simulink model "TotemPoleBoostPFCTestHarnessPlant"  (R2026a)
settings: Solver=ode3  StopTime=0.08  MaxStep=1e-5  AbsTol=1e-3
PreLoadFcn:
  | TotemPoleBoostPFCDefaultInputParameters;
model workspace (MAT data in the model file):
  ConverterKey = "TotemPoleBoostPFC"
undefined symbols (not defined in the file or in its folder): DiscIntNeverNeededParam, totemPoleController, totemPoleDesign
libraries: ee_lib x27, nesl_utility x23, fl_lib x12
(part 1 of 3)
settings Model: Creator=vsolaise  LastModifiedBy=vsolaise
settings SimscapeCC: SimscapeNominalValues="[{\"value\":\"1\",\"unit\":\"A\"},{\"value\":\"1\",\"unit\":\"bar\"},{\"value\":\"1\",\"unit\":\"cm^2\"},{\"value\":\"1\",\"unit\":\"cm^3/s\"},{\"value\":\"1\",\"unit\":\"kJ/kg\"},{\"value\":\"1\",\"unit\":\"kW\"},{\"value\":\"1\",\"unit\":\"l\"},{\"value\":\"1\",\"unit\":\"N\"},{\"value\":\"1\",\"unit\":\"N*m\"},{\"value\":\"1\",\"unit\":\"V\"}]"  SimscapeLogDataHistory=5000.0

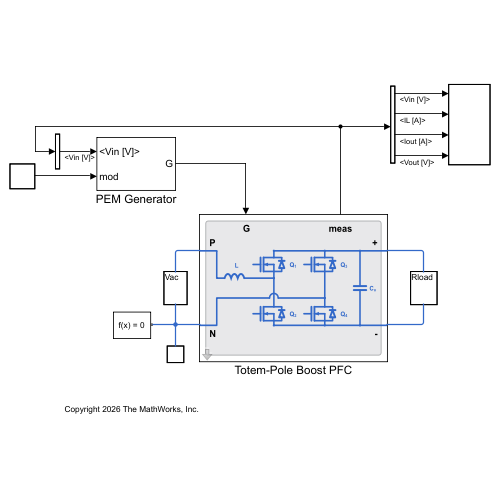
[thumbnail: Simulink's stored preview of the top-level diagram]
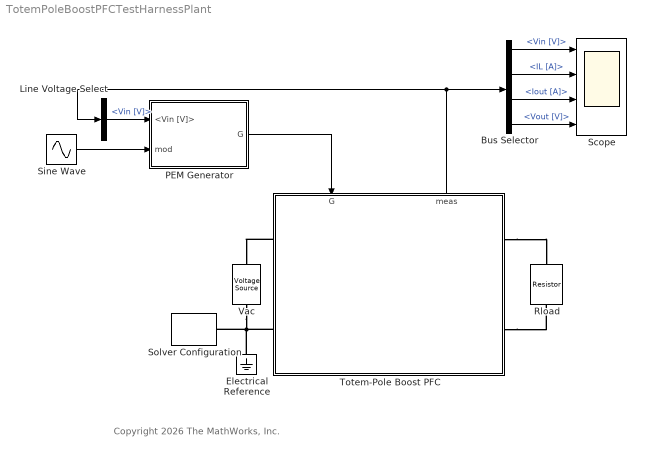
== system TotemPoleBoostPFCTestHarnessPlant ==
  note: Copyright 2026 The MathWorks, Inc.
  Bus Selector : BusSelector  OutputSignals=Vin [V],IL [A],Iout [A],Vout [V]
  Electrical Reference : fl_lib/Electrical/Electrical Elements/Electrical Reference
  Line Voltage Select : BusSelector  OutputSignals=Vin [V]
  PEM Generator : Subsystem
  Rload : fl_lib/Electrical/Electrical Elements/Resistor  R=400 Ohm  i_specify=off  i_priority=None  i=0 A  i_nominal_specify=off  i_nominal_value=1  i_nominal_unit=A  v_specify=off  v_priority=None  v=0 V  v_nominal_specify=off  v_nominal_value=1  v_nominal_unit=V
  Scope : Scope  NumInputPorts=4
      settings: ActiveDisplayString=4  Title=Output Voltage (A)  ActiveDisplayYMinimum=-130.93965530314475  ActiveDisplayYMaximum=1373.5135381119831
  Sine Wave : Sin  Amplitude=0.8  Frequency=50*2*pi  Phase=0.44*pi/180  SampleTime=0
  Solver Configuration : nesl_utility/Solver Configuration  PhysicalDomain=network_engine_domain  SubClassName=solver  LeftPortType=input  RightPortType=generic  Tones=[]  Harmonics=[]  SimulateNoise=off  Profile=off  UseLocalSampling=off  EnableSwitchedLinearOptims=on  FrequencyDomain=off  UseCCode=off  RelTol=0.001  AbsTol=0.001  MinStep=1e-09  ToWorkspace=off  RevertToSquareIcSolve=off  NumHomotopyIterations=100  PhasorMode=off  PhasorModeNumHarmonics=1  ConsistencySolver=NEWTON_XTOL_AFTER_FTOL  CanonicalOrdering=UNORDERED  OptimizeIntermediates=UNOPTIMIZED  IndexReductionMethod=DerivativeReplacement  DoDC=off  ResidualTolerance=1e-09  ConsistencyTolSource=GLOBAL  ConsistencyAbsTol=0.001  ConsistencyRelTol=0.001  ConsistencyTolFactor=0.001  UseLocalSolver=on  LocalSolverChoice=NE_BACKWARD_EULER_ADVANCER  ResolveIndetEquations=on  FunctionEvalNumThread=1  LocalSolverSampleTime=2e-7  DoFixedCost=on  MaxNonlinIter=6  MaxModeIter=2  ComputeImpulses=off  ImpulseIterations=2  LinearAlgebra=auto  LinearAlgebraNumThread=0  EquationFormulation=NE_TIME_EF  DelaysMemoryBudget=1024  AutomaticFiltering=on  FilteringTimeConstant=0.001  PartitionStorageMethod=AS_NEEDED  PartitionMemoryBudget=1024  PartitionMethod=ROBUST  MultibodyUseLocalSolver=off  MultibodyLocalSolverChoice=ODE1  MultibodyLocalSolverSampleTime=0.001
  Totem-Pole Boost PFC : Subsystem  mask(Totem-Pole Boost PFC Converter){modelOption=Simplified, ratedPower=3000, ratedPower_unit=W, VIn=230, VIn_unit=V, FRated=50, FRated_unit=Hz, VOut=400, VOut_unit=V, Fsw=100000, Fsw_unit=Hz, LBoost=2.0742e-4, LBoost_unit=H, RLboost=0.02, RLboost_unit=Ohm, CBoost=1.1937e-3, CBoost_unit=F, Rco=0.01, Rco_unit=Ohm, Vco=400, Vco_unit=V, fastLegDeviceOption=MOSFET (Ideal, Switching) with Thermal, RdsOnFast=0.04, RdsOnFast_unit=Ohm, GdsOffFast=1e-5, GdsOffFast_unit=1/Ohm, VthFast=3, VthFast_unit=V, simTempFast=25, simTempFast_unit=degC, slowLegDeviceOption=MOSFET, slowMOSFETDeviceOption=MOSFET (Ideal, Switching) with Thermal, slowDiodeDeviceOption=Ideal Diode, RdsOnSlow=0.05, RdsOnSlow_unit=Ohm, GdsOffSlow=1e-5, GdsOffSlow_unit=1/Ohm, VthSlow=3, VthSlow_unit=V, simTempSlow=25, simTempSlow_unit=degC, VfSlow=0.6, VfSlow_unit=V, RdSlow=0.01, RdSlow_unit=Ohm, GdSlow=1e-8, GdSlow_unit=1/Ohm, IhSlow=1, IhSlow_unit=A, VfFast=0.8, VfFast_unit=V, RdFast=0.001, RdFast_unit=Ohm, GdFast=1e-5, GdFast_unit=1/Ohm}
      mask prompts: modelOption "Totem-Pole Boost PFC Model Option"; ratedPower "Rated Power"; VIn "AC Input Voltage (RMS)"; FRated "Line Frequency"; VOut "DC Output Voltage"; Fsw "Switching Frequency"; LBoost "Boost Inductance"; RLboost "Inductor resistance"; CBoost "Output Capacitance"; Rco "Capacitor ESR"; Vco "Initial Output Capacitor Voltage"; fastLegDeviceOption "Fast Leg Device"; RdsOnFast "On-State Resistance"; GdsOffFast "Off-State Conductance"; VthFast "Threshold Voltage"; simTempFast "Simulation temperature"; slowLegDeviceOption "Slow Leg Device"; slowMOSFETDeviceOption "MOSFET Device"; slowDiodeDeviceOption "Diode Device"; RdsOnSlow "On-State Resistance (MOSFET)"; GdsOffSlow "Off-State Conductance"; VthSlow "Threshold Voltage"; simTempSlow "Simulation temperature"; VfSlow "Forward Voltage (Diode)"; RdSlow "On Resistance (Diode)"; GdSlow "Off Conductance (Diode)"; IhSlow "Holding current (Ih)"; VfFast "Forward Voltage (Body Diode)"; RdFast "On Resistance (Body Diode)"; GdFast "Off Conductance (Body Diode)"
      mask help: Bridgeless totem-pole boost PFC with fast and slow legs
      mask init:
      | %% Unit conversion: convert displayed values to base SI units
      | convMap = containers.Map( ...
      |     {'W','kW','MW','V','kV','mV','A','mA','F','mF','uF','nF','pF', ...
      |      'H','mH','uH','nH','Ohm','kOhm','mOhm','S','mS','1/Ohm', ...
      |      'Hz','kHz','MHz'}, ...
      |     {1, 1e3, 1e6, 1, 1e3, 1e-3, 1, 1e-3, 1, 1e-3, 1e-6, 1e-9, 1e-12, ...
      |      1, 1e-3, 1e-6, 1e-9, 1, 1e3, 1e-3, 1, 1e-3, 1, ...
      |      1, 1e3, 1e6});
      | 
      | ratedPower_SI = ratedPower * convMap(ratedPower_unit);
      | VIn_SI = VIn * convMap(VIn_unit);
      | FRated_SI = FRated * convMap(FRated_unit);
      | VOut_SI = VOut * convMap(VOut_unit);
      | Fsw_SI = Fsw * convMap(Fsw_unit);
      | LBoost_SI = LBoost * convMap(LBoost_unit);
      | RLboost_SI = RLboost * convMap(RLboost_unit);
      | CBoost_SI = CBoost * convMap(CBoost_unit);
      | Rco_SI = Rco * convMap(Rco_unit);
      | Vco_SI = Vco * convMap(Vco_unit);
      | RdsOnFast_SI = RdsOnFast * convMap(RdsOnFast_unit);
      | GdsOffFast_SI = GdsOffFast * convMap(GdsOffFast_unit);
      | VthFast_SI = VthFast * convMap(VthFast_unit);
      | VfFast_SI = VfFast * convMap(VfFast_unit);
      | RdFast_SI = RdFast * convMap(RdFast_unit);
      | GdFast_SI = GdFast * convMap(GdFast_unit);
      | RdsOnSlow_SI = RdsOnSlow * convMap(RdsOnSlow_unit);
      | GdsOffSlow_SI = GdsOffSlow * convMap(GdsOffSlow_unit);
      | VthSlow_SI = VthSlow * convMap(VthSlow_unit);
      | VfSlow_SI = VfSlow * convMap(VfSlow_unit);
      | RdSlow_SI = RdSlow * convMap(RdSlow_unit);
      | GdSlow_SI = GdSlow * convMap(GdSlow_unit);
      | IhSlow_SI = IhSlow * convMap(IhSlow_unit);
      | 
      | %% Simulation temperature (thermal MOSFET and tabulated diode)
      | % Temperature is an OFFSET unit (K = degC + 273.15), so it cannot use the
      | % multiplicative convMap; convert it explicitly. These Kelvin variables are
      | % read directly by each thermal MOSFET junction-temperature target, by each leg's
      | % Temperature Source, and by the slow-leg tabulated diodes' device simulation
      | % temperature - the only temperature input those diodes have, since they carry no
      | % thermal port.
      | if strcmp(simTempFast_unit, 'degC')
      |     simTempFast_K = simTempFast + 273.15;
      | else
      |     simTempFast_K = simTempFast;
      | end
      | if strcmp(simTempSlow_unit, 'degC')
      |     simTempSlow_K = simTempSlow + 273.15;
      | else
      |     simTempSlow_K = simTempSlow;
      | end
      | 
      | %% Apply variant selection
      | selectTotemPolePFCModelOption(gcb);
      settings: CopyFcn="set_param(gcbh,\"LinkStatus\",\"none\");"  PortSchema="{\"entries\":[{\"content\":{\"sides\":[{\"content\":{\"connectorIds\":[\"LConn1\",\"LConn2\"]},\"type\":\"ConnectorPlacement.EquallySpacedRectSide\",\"uuid\":\"1524dc94-6d10-41c3-9c4d-140b0cbad198\"},{\"content\":{\"connectorIds\":[\"RConn1\",\"RConn2\"],\"side\":\"RIGHT\"},\"type\":\"ConnectorPlacement.EquallySpacedRectSide\",\"uuid\":\"3d33c594-269c-419c-bd3b-3274925b3c44\"},{\"content\":{\"connectorIds\":[\"In1\",\"Out1\"],\"side\":\"TOP\"},\"type\":\"ConnectorPlacement.EquallySpacedRectSide\",\"uuid\":\"36540d5a-957f-45fd-8e0e-0b298bd16df8\"}]},\"type\":\"ConnectorPlacement.EquallySpacedConnector\",\"uuid\":\"4eeec72c-6b37-4cf7-b4fd-97832ebea029\"}],\"packageUris\":[\"http://schema.mathworks.com/mf0/Connector/R2020b\"],\"version\":\"1.0\"}"
      mask Help: web('TotemPoleBoostPFC.html')
      mask TypeOptions modelOption: Simplified | Detailed
      mask Callback modelOption: selectTotemPolePFCModelOption(gcb);
      mask TypeOptions ratedPower_unit: W | kW | MW
      mask TypeOptions VIn_unit: V | kV | mV
      mask TypeOptions FRated_unit: Hz | kHz
      mask TypeOptions VOut_unit: V | kV | mV
      mask TypeOptions Fsw_unit: Hz | kHz | MHz
      mask TypeOptions LBoost_unit: H | mH | uH
      mask TypeOptions RLboost_unit: Ohm | kOhm | mOhm
      mask TypeOptions CBoost_unit: F | mF | uF | nF
      mask TypeOptions Rco_unit: Ohm | kOhm | mOhm
      mask TypeOptions Vco_unit: V | kV | mV
      mask TypeOptions fastLegDeviceOption: Ideal Switch | MOSFET (Ideal, Switching) with Thermal
      mask Callback fastLegDeviceOption: selectTotemPolePFCFastLeg(gcb);
      mask TypeOptions RdsOnFast_unit: Ohm | kOhm | mOhm
      mask TypeOptions GdsOffFast_unit: 1/Ohm | S | mS
      mask TypeOptions VthFast_unit: V | kV | mV
      mask TypeOptions simTempFast_unit: degC | K
      mask TypeOptions slowLegDeviceOption: Diode | MOSFET | Thyristor
      mask Callback slowLegDeviceOption: selectTotemPolePFCSlowLeg(gcb);
      mask TypeOptions slowMOSFETDeviceOption: Ideal Switch | MOSFET (Ideal, Switching) with Thermal
      mask Callback slowMOSFETDeviceOption: selectTotemPoleSlowMOSFETDevice(gcb);
      mask TypeOptions slowDiodeDeviceOption: Ideal Diode | Tabulated Diode
      mask Callback slowDiodeDeviceOption: selectTotemPoleSlowDiodeDevice(gcb);
      mask TypeOptions RdsOnSlow_unit: Ohm | kOhm | mOhm
      mask TypeOptions GdsOffSlow_unit: 1/Ohm | S | mS
      mask TypeOptions VthSlow_unit: V | kV | mV
      mask TypeOptions simTempSlow_unit: degC | K
      mask TypeOptions VfSlow_unit: V | kV | mV
      mask TypeOptions RdSlow_unit: Ohm | kOhm | mOhm
      mask TypeOptions GdSlow_unit: 1/Ohm | S | mS
      mask TypeOptions IhSlow_unit: A
      mask TypeOptions VfFast_unit: V | kV | mV
      mask TypeOptions RdFast_unit: Ohm | kOhm | mOhm
      mask TypeOptions GdFast_unit: 1/Ohm | S | mS
      mask DialogControl Totem_PoleBoostPFCConverterParameters Prompt: Totem-Pole Boost PFC Converter Parameters
      mask DialogControl FastLegDevice Prompt: Fast Leg Device
      mask DialogControl openFastMOSFETMask Prompt: Open MOSFET block mask
      mask DialogControl openFastMOSFETMask Callback: openTotemPoleDeviceMask(gcb, 'fastThermalMOSFET');
      mask DialogControl applyFastMOSFETParam Prompt: Apply parameters to all fast leg MOSFET blocks
      mask DialogControl applyFastMOSFETParam Callback: applyTotemPoleFastMOSFETParameters(gcb);
      mask DialogControl SlowLegDevice Prompt: Slow Leg Device
      mask DialogControl openSlowMOSFETMask Prompt: Open MOSFET block mask
      mask DialogControl openSlowMOSFETMask Callback: openTotemPoleDeviceMask(gcb, 'slowThermalMOSFET');
      mask DialogControl applySlowMOSFETParam Prompt: Apply parameters to all slow leg MOSFET blocks
      mask DialogControl applySlowMOSFETParam Callback: applyTotemPoleSlowMOSFETParameters(gcb);
      mask DialogControl openSlowDiodeMask Prompt: Open Diode block mask
      mask DialogControl openSlowDiodeMask Callback: openTotemPoleDeviceMask(gcb, 'slowTabulatedDiode');
      mask DialogControl applySlowDiodeParam Prompt: Apply parameters to all slow leg Diode blocks
      mask DialogControl applySlowDiodeParam Callback: applyTotemPoleSlowDiodeParameters(gcb);
      mask DialogControl ExportPanel Prompt: Export to Unmasked Subsystem
      mask DialogControl ExportInfo Prompt: To customize the converter, export it as an unmasked subsystem with the active variant flattened - a standalone, fully-editable circuit plus a parameter file. Requires the "Variant Manager for Simulink" add-on.
      mask DialogControl exportToModel Prompt: Export
      mask DialogControl exportToModel Callback: exportConverterModelFromMask(gcb);
      mask Display:
      | slowLeg = get_param(gcb, 'slowLegDeviceOption');
      | if strcmp(slowLeg, 'Diode')
      |     image('TotemPoleDiodeIcon.svg');
      | elseif strcmp(slowLeg, 'Thyristor')
      |     image('TotemPoleThyristorIcon.svg');
      | else
      |     image('TotemPoleMOSFETIcon.svg');
      | end
  Vac : ee_lib/Sources/Voltage Source  dc_voltage=0 V  ac_voltage=230*sqrt(2) V  ac_shift=0 rad  ac_frequency=50 Hz  noise_mode=ee.enum.sources.noise.Disabled  PSD=0 V^2/Hz  sample_time=1e-3 s  repeatability=ee.enum.sources.repeatability.NotRepeatable  user_seed=0  auto_seed=3037630589  i_specify=off  i_priority=None  i=0 A  i_nominal_specify=off  i_nominal_value=1  i_nominal_unit=A  v_specify=off  v_priority=None  v=0 V  v_nominal_specify=off  v_nominal_value=1  v_nominal_unit=V
  wires:
  Totem-Pole Boost PFC/1(meas) -> Bus Selector/1, Line Voltage Select/1
  Bus Selector/1 -> Scope/1  "<Vin [V]>"
  Bus Selector/2 -> Scope/2  "<IL [A]>"
  Bus Selector/3 -> Scope/3  "<Iout [A]>"
  Bus Selector/4 -> Scope/4  "<Vout [V]>"
  Line Voltage Select/1 -> PEM Generator/1(<Vin [V]>)  "<Vin [V]>"
  PEM Generator/1(G) -> Totem-Pole Boost PFC/1(G)
  Sine Wave/1 -> PEM Generator/2(mod)
  connections:
  Totem-Pole Boost PFC/LConn1 -- Vac/LConn1
  Vac/RConn1 -- Electrical Reference/LConn1 -- Solver Configuration/RConn1 -- Totem-Pole Boost PFC/LConn2
  Totem-Pole Boost PFC/RConn1 -- Rload/LConn1
  Totem-Pole Boost PFC/RConn2 -- Rload/RConn1

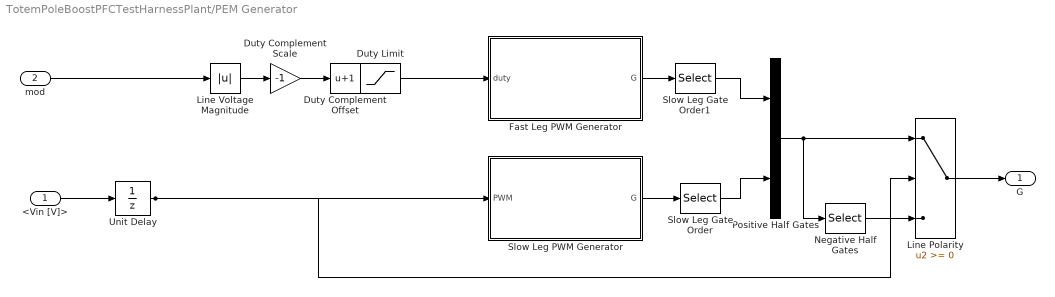
== system TotemPoleBoostPFCTestHarnessPlant/PEM Generator ==
  <Vin [V]> : Inport
  mod : Inport  Port=2
  Duty Complement Offset : Bias  Bias=1  SaturateOnIntegerOverflow=off
  Duty Complement Scale : Gain  Gain=-1
  Duty Limit : Saturate  UpperLimit=totemPoleController.dutyMax  LowerLimit=totemPoleController.dutyMin
  Fast Leg PWM Generator : Subsystem  mask(Half Bridge PWM Generator){solverMode=Variable-step (continuous), Ts=1e-8, Fsw=totemPoleDesign.switchingFrequency.value, Tdead=totemPoleController.fastLegDeadTime, gateVoltageOn=totemPoleController.gateVoltageOn, gateVoltageOff=totemPoleController.gateVoltageOff}
      mask prompts: solverMode "Solver mode"; Ts "Sample time (s)"; Fsw "Switching frequency (Hz)"; Tdead "Dead time (s)"; gateVoltageOn "Gate ON voltage (V)"; gateVoltageOff "Gate OFF voltage (V)"
      mask help:
      | This block generates half-bridge PWM gate signals with a dead time from a commanded duty cycle.
      |
      | For a variable-step solver, set Solver mode to Variable-step (continuous). For a fixed-step solver, set Solver mode to Fixed-step (discrete) and set Sample time to a positive value.
      mask init:
      | % Solver mode. Switch every sawtooth ramp in this block between its continuous
      | % and its discrete implementation, and show the sample time only when it is used.
      | pwmGeneratorBlock = gcb;
      | if strcmp(get_param(pwmGeneratorBlock, 'solverMode'), 'Fixed-step (discrete)')
      |     pwmGeneratorRampChoice = 'FixedStep';
      |     pwmGeneratorSampleTimeVisibility = 'on';
      | else
      |     pwmGeneratorRampChoice = 'VariableStep';
      |     pwmGeneratorSampleTimeVisibility = 'off';
      | end
      | 
      | % A block may hold more than one ramp, at any depth, so the ramps are found by the
      | % "Ramp Mode" suffix on their names rather than by one fixed path. The match filter
      | % keeps every variant choice in the search, which is also what silences the
      | % find_system default-variants warning.
      | pwmGeneratorRamps = find_system(pwmGeneratorBlock, ...
      |     'MatchFilter', @Simulink.match.allVariants, 'LookUnderMasks', 'all', ...
      |     'FollowLinks', 'on', 'Regexp', 'on', 'BlockType', 'SubSystem', ...
      |     'Name', 'Ramp Mode$');
      | for pwmGeneratorRampIndex = 1:numel(pwmGeneratorRamps)
      |     set_param(pwmGeneratorRamps{pwmGeneratorRampIndex}, ...
      |         'LabelModeActiveChoice', pwmGeneratorRampChoice);
      | end
      | 
      | % Only the discrete ramp declares a rate, so the sample time is hidden in the
      | % continuous mode. The guard keeps the code silent on a mask still being built.
      | pwmGeneratorMask = Simulink.Mask.get(pwmGeneratorBlock);
      | pwmGeneratorSampleTime = pwmGeneratorMask.getParameter('Ts');
      | if ~isempty(pwmGeneratorSampleTime)
      |     pwmGeneratorSampleTime.Visible = pwmGeneratorSampleTimeVisibility;
      | end
      mask Help: web('HalfBridgePWMGenerator.html')
      mask TypeOptions solverMode: Variable-step (continuous) | Fixed-step (discrete)
      mask Callback solverMode:
      | % Solver mode. Switch every sawtooth ramp in this block between its continuous
      | % and its discrete implementation, and show the sample time only when it is used.
      | pwmGeneratorBlock = gcb;
      | if strcmp(get_param(pwmGeneratorBlock, 'solverMode'), 'Fixed-step (discrete)')
      |     pwmGeneratorRampChoice = 'FixedStep';
      |     pwmGeneratorSampleTimeVisibility = 'on';
      | else
      |     pwmGeneratorRampChoice = 'VariableStep';
      |     pwmGeneratorSampleTimeVisibility = 'off';
      | end
      | 
      | % A block may hold more than one ramp, at any depth, so the ramps are found by the
      | % "Ramp Mode" suffix on their names rather than by one fixed path. The match filter
      | % keeps every variant choice in the search, which is also what silences the
      | % find_system default-variants warning.
      | pwmGeneratorRamps = find_system(pwmGeneratorBlock, ...
      |     'MatchFilter', @Simulink.match.allVariants, 'LookUnderMasks', 'all', ...
      |     'FollowLinks', 'on', 'Regexp', 'on', 'BlockType', 'SubSystem', ...
      |     'Name', 'Ramp Mode$');
      | for pwmGeneratorRampIndex = 1:numel(pwmGeneratorRamps)
      |     set_param(pwmGeneratorRamps{pwmGeneratorRampIndex}, ...
      |         'LabelModeActiveChoice', pwmGeneratorRampChoice);
      | end
      | 
      | % Only the discrete ramp declares a rate, so the sample time is hidden in the
      | % continuous mode. The guard keeps the code silent on a mask still being built.
      | pwmGeneratorMask = Simulink.Mask.get(pwmGeneratorBlock);
      | pwmGeneratorSampleTime = pwmGeneratorMask.getParameter('Ts');
      | if ~isempty(pwmGeneratorSampleTime)
      |     pwmGeneratorSampleTime.Visible = pwmGeneratorSampleTimeVisibility;
      | end
      mask DialogControl DescTextVar Prompt:
      | This block generates half-bridge PWM gate signals with a dead time from a commanded duty cycle.
      | 
      | For a variable-step solver, set Solver mode to Variable-step (continuous). For a fixed-step solver, set Solver mode to Fixed-step (discrete) and set Sample time to a positive value.
      mask DialogControl SolverPanel Prompt: Solver Settings
      mask DialogControl SwitchingPanel Prompt: Switching Parameters
      mask DialogControl GateDrivePanel Prompt: Gate Drive
  Line Polarity : Switch  SaturateOnIntegerOverflow=off  InputSameDT=off
  Line Voltage Magnitude : Abs  SaturateOnIntegerOverflow=off
  Negative Half Gates : Selector  InputPortWidth=4  IndexOptions=Index vector (dialog)  Indices=[2 1 3 4]  OutputSizes=1
  Positive Half Gates : Mux  Inputs=2
  Slow Leg Gate Order : Selector  InputPortWidth=2  IndexOptions=Index vector (dialog)  Indices=[2 1]  OutputSizes=1
  Slow Leg Gate Order1 : Selector  InputPortWidth=2  IndexOptions=Index vector (dialog)  Indices=[2 1]  OutputSizes=1
  Slow Leg PWM Generator : Subsystem  mask(Complementary PWM Generator){solverMode=Variable-step (continuous), Ts=1e-8, Tdead=totemPoleController.slowLegTurnOnDelay, inputLogicThreshold=0, gateVoltageOn=totemPoleController.gateVoltageOn, gateVoltageOff=totemPoleController.gateVoltageOff}
      mask prompts: solverMode "Solver mode"; Ts "Sample time (s)"; Tdead "Dead time (s)"; inputLogicThreshold "Input logic threshold (V)"; gateVoltageOn "Gate ON voltage (V)"; gateVoltageOff "Gate OFF voltage (V)"
      mask help:
      | This block splits one PWM signal into a complementary gate pair with a dead time.
      |
      | For a variable-step solver, set Solver mode to Variable-step (continuous). For a fixed-step solver, set Solver mode to Fixed-step (discrete) and set Sample time to a positive value.
      mask init: same as TotemPoleBoostPFCTestHarnessPlant/PEM Generator/Fast Leg PWM Generator
      mask Help: web('ComplementaryPWMGenerator.html')
      mask TypeOptions solverMode: Variable-step (continuous) | Fixed-step (discrete)
      mask Callback solverMode:
      | % Solver mode. Switch every sawtooth ramp in this block between its continuous
      | % and its discrete implementation, and show the sample time only when it is used.
      | pwmGeneratorBlock = gcb;
      | if strcmp(get_param(pwmGeneratorBlock, 'solverMode'), 'Fixed-step (discrete)')
      |     pwmGeneratorRampChoice = 'FixedStep';
      |     pwmGeneratorSampleTimeVisibility = 'on';
      | else
      |     pwmGeneratorRampChoice = 'VariableStep';
      |     pwmGeneratorSampleTimeVisibility = 'off';
      | end
      | 
      | % A block may hold more than one ramp, at any depth, so the ramps are found by the
      | % "Ramp Mode" suffix on their names rather than by one fixed path. The match filter
      | % keeps every variant choice in the search, which is also what silences the
      | % find_system default-variants warning.
      | pwmGeneratorRamps = find_system(pwmGeneratorBlock, ...
      |     'MatchFilter', @Simulink.match.allVariants, 'LookUnderMasks', 'all', ...
      |     'FollowLinks', 'on', 'Regexp', 'on', 'BlockType', 'SubSystem', ...
      |     'Name', 'Ramp Mode$');
      | for pwmGeneratorRampIndex = 1:numel(pwmGeneratorRamps)
      |     set_param(pwmGeneratorRamps{pwmGeneratorRampIndex}, ...
      |         'LabelModeActiveChoice', pwmGeneratorRampChoice);
      | end
      | 
      | % Only the discrete ramp declares a rate, so the sample time is hidden in the
      | % continuous mode. The guard keeps the code silent on a mask still being built.
      | pwmGeneratorMask = Simulink.Mask.get(pwmGeneratorBlock);
      | pwmGeneratorSampleTime = pwmGeneratorMask.getParameter('Ts');
      | if ~isempty(pwmGeneratorSampleTime)
      |     pwmGeneratorSampleTime.Visible = pwmGeneratorSampleTimeVisibility;
      | end
      mask DialogControl DescTextVar Prompt:
      | This block splits one PWM signal into a complementary gate pair with a dead time.
      | 
      | For a variable-step solver, set Solver mode to Variable-step (continuous). For a fixed-step solver, set Solver mode to Fixed-step (discrete) and set Sample time to a positive value.
      mask DialogControl SolverPanel Prompt: Solver Settings
      mask DialogControl SwitchingPanel Prompt: Switching Parameters
      mask DialogControl GateDrivePanel Prompt: Gate Drive
  Unit Delay : UnitDelay  SampleTime=-1
  G : Outport
  wires:
  Slow Leg Gate Order/1 -> Positive Half Gates/2
  Negative Half Gates/1 -> Line Polarity/3
  Duty Limit/1 -> Fast Leg PWM Generator/1(duty)
  Line Polarity/1 -> G/1
  Fast Leg PWM Generator/1(G) -> Slow Leg Gate Order1/1
  <Vin [V]>/1 -> Unit Delay/1
  Slow Leg PWM Generator/1(G) -> Slow Leg Gate Order/1
  Positive Half Gates/1 -> Negative Half Gates/1, Line Polarity/1
  mod/1 -> Line Voltage Magnitude/1
  Slow Leg Gate Order1/1 -> Positive Half Gates/1
  Line Voltage Magnitude/1 -> Duty Complement Scale/1
  Duty Complement Scale/1 -> Duty Complement Offset/1
  Duty Complement Offset/1 -> Duty Limit/1
  Unit Delay/1 -> Line Polarity/2, Slow Leg PWM Generator/1(PWM)

== system TotemPoleBoostPFCTestHarnessPlant/Totem-Pole Boost PFC ==
  G : Inport
  TotemPoleBoostPFCVariant : Subsystem  Variant=on  VariantControlMode=label  LabelModeActiveChoice=SimplifiedModel
  P : PMIOPort  Side=Left
  N : PMIOPort  Port=2  Side=Left
  + : PMIOPort  Port=3  Side=Right
  - : PMIOPort  Port=4  Side=Right
  meas : Outport
  wires:
  G/1 -> TotemPoleBoostPFCVariant/1(G)
  TotemPoleBoostPFCVariant/1(meas) -> meas/1
  connections:
  P/RConn1 -- TotemPoleBoostPFCVariant/LConn1
  N/RConn1 -- TotemPoleBoostPFCVariant/LConn2
  TotemPoleBoostPFCVariant/RConn1 -- +/RConn1
  TotemPoleBoostPFCVariant/RConn2 -- -/RConn1

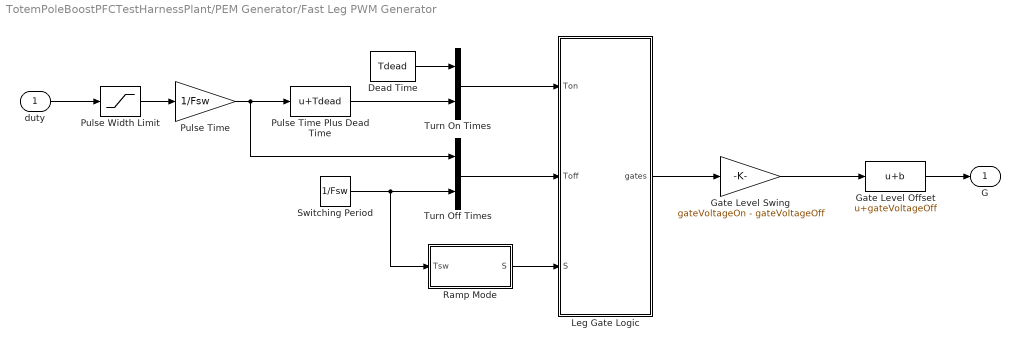
== system TotemPoleBoostPFCTestHarnessPlant/PEM Generator/Fast Leg PWM Generator ==
  duty : Inport
  Dead Time : Constant  Value=Tdead
  Gate Level Offset : Bias  Bias=gateVoltageOff
  Gate Level Swing : Gain  Gain=gateVoltageOn - gateVoltageOff
  Leg Gate Logic : Subsystem
  Pulse Time : Gain  Gain=1/Fsw
  Pulse Time Plus Dead Time : Bias  Bias=Tdead
  Pulse Width Limit : Saturate  UpperLimit=1 - Tdead*Fsw  LowerLimit=Tdead*Fsw
  Ramp Mode : Subsystem  Variant=on  VariantControlMode=label  LabelModeActiveChoice=VariableStep
  Switching Period : Constant  Value=1/Fsw
  Turn Off Times : Mux  Inputs=2
  Turn On Times : Mux  Inputs=2
  G : Outport
  wires:
  Gate Level Offset/1 -> G/1
  Leg Gate Logic/1(gates) -> Gate Level Swing/1
  Ramp Mode/1(S) -> Leg Gate Logic/3(S)
  Turn Off Times/1 -> Leg Gate Logic/2(Toff)
  Turn On Times/1 -> Leg Gate Logic/1(Ton)
  Gate Level Swing/1 -> Gate Level Offset/1
  Switching Period/1 -> Ramp Mode/1(Tsw), Turn Off Times/2
  Pulse Time Plus Dead Time/1 -> Turn On Times/2
  Dead Time/1 -> Turn On Times/1
  Pulse Time/1 -> Turn Off Times/1, Pulse Time Plus Dead Time/1
  Pulse Width Limit/1 -> Pulse Time/1
  duty/1 -> Pulse Width Limit/1

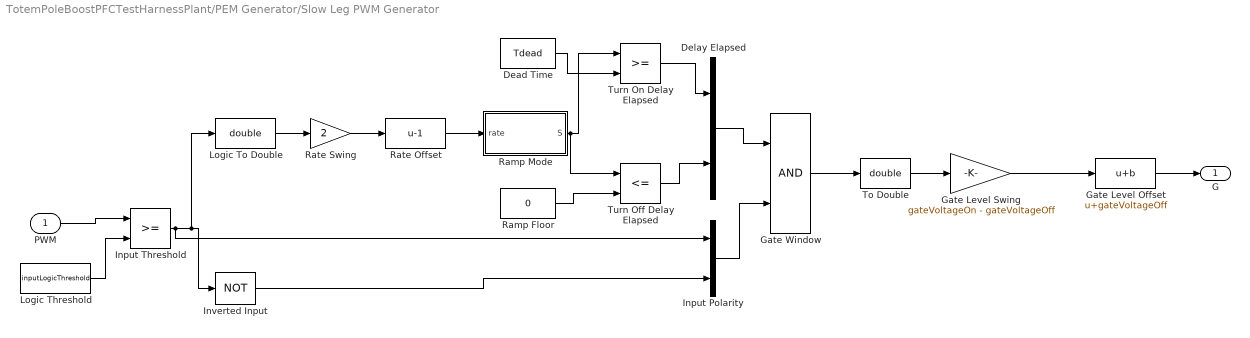
== system TotemPoleBoostPFCTestHarnessPlant/PEM Generator/Slow Leg PWM Generator ==
  PWM : Inport
  Dead Time : Constant  Value=Tdead
  Delay Elapsed : Mux  Inputs=2
  Gate Level Offset : Bias  Bias=gateVoltageOff
  Gate Level Swing : Gain  Gain=gateVoltageOn - gateVoltageOff
  Gate Window : Logic
  Input Polarity : Mux  Inputs=2
  Input Threshold : RelationalOperator
  Inverted Input : Logic  Operator=NOT  Inputs=1
  Logic Threshold : Constant  Value=inputLogicThreshold
  Logic To Double : DataTypeConversion  OutDataTypeStr=double
  Ramp Floor : Constant  Value=0
  Ramp Mode : Subsystem  Variant=on  VariantControlMode=label  LabelModeActiveChoice=VariableStep
  Rate Offset : Bias  Bias=-1
  Rate Swing : Gain  Gain=2
  To Double : DataTypeConversion  OutDataTypeStr=double
  Turn Off Delay Elapsed : RelationalOperator  Operator=<=
  Turn On Delay Elapsed : RelationalOperator
  G : Outport
  wires:
  Gate Level Offset/1 -> G/1
  To Double/1 -> Gate Level Swing/1
  Gate Window/1 -> To Double/1
  Input Polarity/1 -> Gate Window/2
  Delay Elapsed/1 -> Gate Window/1
  Turn Off Delay Elapsed/1 -> Delay Elapsed/2
  Turn On Delay Elapsed/1 -> Delay Elapsed/1
  Ramp Floor/1 -> Turn Off Delay Elapsed/2
  Dead Time/1 -> Turn On Delay Elapsed/2
  Ramp Mode/1(S) -> Turn Off Delay Elapsed/1, Turn On Delay Elapsed/1
  Rate Offset/1 -> Ramp Mode/1(rate)
  Rate Swing/1 -> Rate Offset/1
  Logic To Double/1 -> Rate Swing/1
  Inverted Input/1 -> Input Polarity/2
  Input Threshold/1 -> Inverted Input/1, Logic To Double/1, Input Polarity/1
  Logic Threshold/1 -> Input Threshold/2
  PWM/1 -> Input Threshold/1
  Gate Level Swing/1 -> Gate Level Offset/1

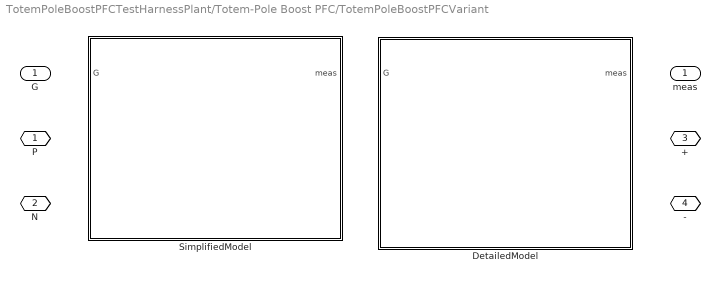
== system TotemPoleBoostPFCTestHarnessPlant/Totem-Pole Boost PFC/TotemPoleBoostPFCVariant ==
  G : Inport
  DetailedModel : Subsystem  VariantControl=DetailedModel
  SimplifiedModel : Subsystem  VariantControl=SimplifiedModel
  P : PMIOPort  Side=Left
  N : PMIOPort  Port=2  Side=Left
  + : PMIOPort  Port=3  Side=Right
  - : PMIOPort  Port=4  Side=Right
  meas : Outport

== system TotemPoleBoostPFCTestHarnessPlant/PEM Generator/Fast Leg PWM Generator/Leg Gate Logic ==
  Ton : Inport
  Toff : Inport  Port=2
  S : Inport  Port=3
  After Turn Off : RelationalOperator
  After Turn On : RelationalOperator
  Pulse Window : Logic  Operator=XOR
  To Double : DataTypeConversion  OutDataTypeStr=double
  gates : Outport
  wires:
  To Double/1 -> gates/1
  Pulse Window/1 -> To Double/1
  After Turn Off/1 -> Pulse Window/2
  After Turn On/1 -> Pulse Window/1
  S/1 -> After Turn On/1, After Turn Off/1
  Toff/1 -> After Turn Off/2
  Ton/1 -> After Turn On/2

== system TotemPoleBoostPFCTestHarnessPlant/PEM Generator/Fast Leg PWM Generator/Ramp Mode ==
  Tsw : Inport
  FixedStep : Subsystem  VariantControl=FixedStep
  VariableStep : Subsystem  VariantControl=VariableStep
  S : Outport

== system TotemPoleBoostPFCTestHarnessPlant/PEM Generator/Slow Leg PWM Generator/Ramp Mode ==
  rate : Inport
  FixedStep : Subsystem  VariantControl=FixedStep
  VariableStep : Subsystem  VariantControl=VariableStep
  S : Outport

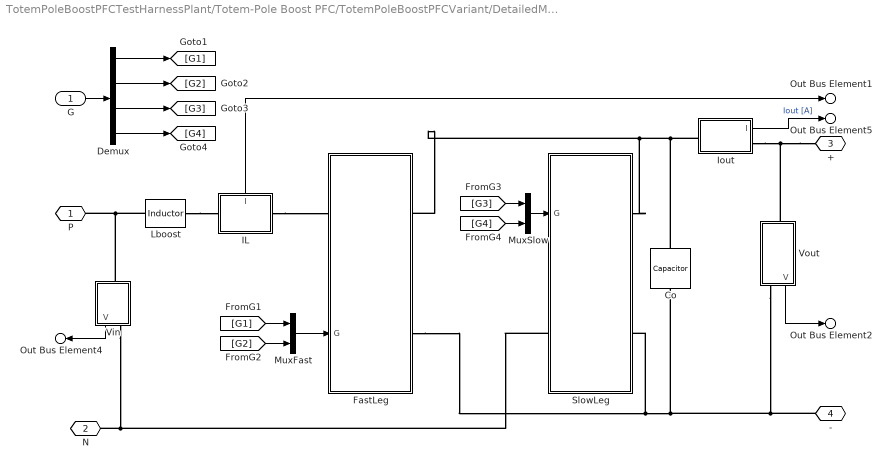
== system TotemPoleBoostPFCTestHarnessPlant/Totem-Pole Boost PFC/TotemPoleBoostPFCVariant/DetailedModel ==
  G : Inport
  Co : ee_lib/Passive/Capacitor  cap_option=ee.enum.passive.capacitor.capOption.const  c=CBoost_SI F  Cvec=[1e-05, 1e-06] F  Vvec=[0, 10] V  CV_table_symmetry=ee.enum.passive.capacitor.tableSymmetry.yes  f_vec=[1, 10] kHz  DFext_vec=[.8, 1.2]  enable_C_tol=ee.enum.toleranceApplication.none  averaging_period=0 s  C_tol=5  tol_distribution=ee.enum.toleranceDistribution.uniform  nSigma=4  r=Rco_SI Ohm  g=0 1/Ohm  enable_operating_limits=ee.enum.enable.no  operating_limit_action=ee.enum.passive.reportOpLim.warn  max_working_voltage_range=[-25, 25] V  power_rating=1 W  maxTemperature=85 degC  thermalEnable=false  thermalMass=1 J/K  i_specify=off  i_priority=None  i=0 A  i_nominal_specify=off  i_nominal_value=1  i_nominal_unit=A  v_specify=off  v_priority=None  v=0 V  v_nominal_specify=off  v_nominal_value=1  v_nominal_unit=V  vc_specify=on  vc_priority=High  vc=Vco_SI V  vc_nominal_specify=off  vc_nominal_value=1  vc_nominal_unit=V  T_specify=off  T_priority=None  T=298.15 K  T_nominal_specify=off  T_nominal_value=1  T_nominal_unit=K
  Demux : Demux
  FastLeg : Subsystem  Variant=on  VariantControlMode=label  LabelModeActiveChoice=SwitchingMOSFETwithThermal
      settings: PortSchema="{\"entries\":[{\"content\":{\"sides\":[{\"content\":{\"connectorIds\":[\"LConn1\",\"In1\"]},\"type\":\"ConnectorPlacement.EquallySpacedRectSide\",\"uuid\":\"77e2eceb-8f65-4ff8-b710-02732b9bb145\"},{\"content\":{\"connectorIds\":[\"RConn1\",\"RConn2\"],\"side\":\"RIGHT\"},\"type\":\"ConnectorPlacement.EquallySpacedRectSide\",\"uuid\":\"bfc7df5d-eb60-4c5b-86be-68c51cd3b8c3\"},{\"content\":{\"side\":\"TOP\"},\"type\":\"ConnectorPlacement.EquallySpacedRectSide\",\"uuid\":\"613efa33-60b7-4b5b-9311-a6c7287e5913\"}]},\"type\":\"ConnectorPlacement.EquallySpacedConnector\",\"uuid\":\"12746f96-860a-4c97-9f60-ace4c102aa63\"}],\"packageUris\":[\"http://schema.mathworks.com/mf0/Connector/R2020b\"],\"version\":\"1.0\"}"
  IL : Subsystem
      settings: PortSchema="{\"entries\":[{\"content\":{\"sides\":[{\"content\":{\"connectorIds\":[\"LConn1\"]},\"type\":\"ConnectorPlacement.EquallySpacedRectSide\",\"uuid\":\"80632e7e-66fe-49c8-894c-61cf7358e53a\"},{\"content\":{\"connectorIds\":[\"RConn1\"],\"side\":\"RIGHT\"},\"type\":\"ConnectorPlacement.EquallySpacedRectSide\",\"uuid\":\"7fb991d4-0257-47fa-8c16-238ff3f2e60c\"},{\"content\":{\"connectorIds\":[\"Out1\"],\"side\":\"TOP\"},\"type\":\"ConnectorPlacement.EquallySpacedRectSide\",\"uuid\":\"a2cf4f5e-7cb3-4577-a513-817a4fd9f07d\"}]},\"type\":\"ConnectorPlacement.EquallySpacedConnector\",\"uuid\":\"e3fac4ca-b917-4eeb-beb4-75837a4782c1\"}],\"packageUris\":[\"http://schema.mathworks.com/mf0/Connector/R2020b\"],\"version\":\"1.0\"}"
      mask Display: disp('I')
  Iout : Subsystem
      mask Display: disp('I')
  Lboost : ee_lib/Passive/Inductor  l=LBoost_SI H  enable_L_tol=ee.enum.toleranceApplication.none  L_tol=20  tol_distribution=ee.enum.toleranceDistribution.uniform  nSigma=4  r=RLboost_SI Ohm  g=1e-9 1/Ohm  enable_operating_limits=ee.enum.enable.no  operating_limit_action=ee.enum.passive.reportOpLim.warn  max_working_current=1 A  power_rating=1 W  i_L_specify=off  i_L_priority=High  i_L=0 A  i_L_nominal_specify=off  i_L_nominal_value=1  i_L_nominal_unit=A
  MuxFast : Mux  Inputs=2
  MuxSlow : Mux  Inputs=2
  SlowLeg : Subsystem  Variant=on  VariantControlMode=label  LabelModeActiveChoice=MOSFET
  Vin : Subsystem
      mask Display: disp('V')
  Vout : Subsystem
      settings: PortSchema="{\"entries\":[{\"content\":{\"sides\":[{\"content\":{\"connectorIds\":[\"LConn1\"]},\"type\":\"ConnectorPlacement.EquallySpacedRectSide\",\"uuid\":\"80632e7e-66fe-49c8-894c-61cf7358e53a\"},{\"content\":{\"connectorIds\":[\"RConn1\",\"Out1\"],\"side\":\"RIGHT\"},\"type\":\"ConnectorPlacement.EquallySpacedRectSide\",\"uuid\":\"7fb991d4-0257-47fa-8c16-238ff3f2e60c\"},{\"content\":{\"side\":\"TOP\"},\"type\":\"ConnectorPlacement.EquallySpacedRectSide\",\"uuid\":\"a2cf4f5e-7cb3-4577-a513-817a4fd9f07d\"}]},\"type\":\"ConnectorPlacement.EquallySpacedConnector\",\"uuid\":\"e3fac4ca-b917-4eeb-beb4-75837a4782c1\"}],\"packageUris\":[\"http://schema.mathworks.com/mf0/Connector/R2020b\"],\"version\":\"1.0\"}"
      mask Display: disp('V')
  P : PMIOPort  Side=Left
  N : PMIOPort  Port=2  Side=Left
  + : PMIOPort  Port=3  Side=Right
  - : PMIOPort  Port=4  Side=Right
  Out Bus Element1 : Outport  PortName=meas  Element=IL [A]
  Out Bus Element2 : Outport  PortName=meas  Element=Vout [V]
  Out Bus Element4 : Outport  PortName=meas  Element=Vin [V]
  Out Bus Element5 : Outport  PortName=meas  Element=Iout [A]
  wires:
  G/1 -> Demux/1
  Demux/4 -> [G4]
  Demux/3 -> [G3]
  Demux/2 -> [G2]
  Demux/1 -> [G1]
  Vout/1(V) -> Out Bus Element2/1
  Iout/1(I) -> Out Bus Element5/1  "Iout [A]"
  IL/1(I) -> Out Bus Element1/1
  [G4] -> MuxSlow/2
  [G3] -> MuxSlow/1
  MuxSlow/1 -> SlowLeg/1(G)
  Vin/1(V) -> Out Bus Element4/1
  [G2] -> MuxFast/2
  [G1] -> MuxFast/1
  MuxFast/1 -> FastLeg/1(G)
  connections:
  Vout/RConn1 -- -/RConn1 -- Co/RConn1 -- FastLeg/RConn2 -- SlowLeg/RConn2
  IL/RConn1 -- FastLeg/LConn1
  +/RConn1 -- Vout/LConn1 -- Iout/RConn1
  N/RConn1 -- SlowLeg/LConn1 -- Vin/RConn1
  Lboost/RConn1 -- IL/LConn1
  Iout/LConn1 -- Co/LConn1 -- FastLeg/RConn1 -- SlowLeg/RConn1
  Vin/LConn1 -- P/RConn1 -- Lboost/LConn1

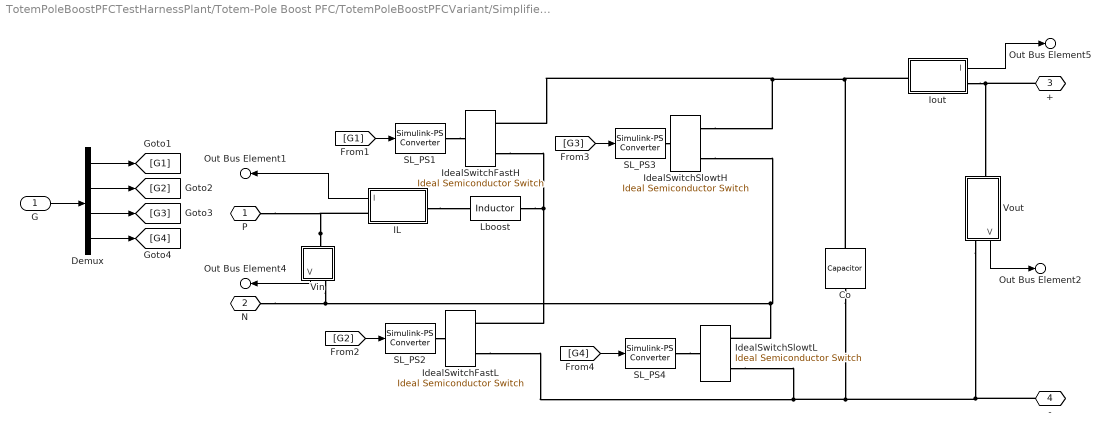
== system TotemPoleBoostPFCTestHarnessPlant/Totem-Pole Boost PFC/TotemPoleBoostPFCVariant/SimplifiedModel ==
  G : Inport
  Co : ee_lib/Passive/Capacitor  cap_option=ee.enum.passive.capacitor.capOption.const  c=CBoost_SI F  Cvec=[1e-05, 1e-06] F  Vvec=[0, 10] V  CV_table_symmetry=ee.enum.passive.capacitor.tableSymmetry.yes  f_vec=[1, 10] kHz  DFext_vec=[.8, 1.2]  enable_C_tol=ee.enum.toleranceApplication.none  averaging_period=0 s  C_tol=5  tol_distribution=ee.enum.toleranceDistribution.uniform  nSigma=4  r=Rco_SI Ohm  g=0 1/Ohm  enable_operating_limits=ee.enum.enable.no  operating_limit_action=ee.enum.passive.reportOpLim.warn  max_working_voltage_range=[-25, 25] V  power_rating=1 W  maxTemperature=85 degC  thermalEnable=false  thermalMass=1 J/K  i_specify=off  i_priority=None  i=0 A  i_nominal_specify=off  i_nominal_value=1  i_nominal_unit=A  v_specify=off  v_priority=None  v=0 V  v_nominal_specify=off  v_nominal_value=1  v_nominal_unit=V  vc_specify=on  vc_priority=High  vc=Vco_SI V  vc_nominal_specify=off  vc_nominal_value=1  vc_nominal_unit=V  T_specify=off  T_priority=None  T=298.15 K  T_nominal_specify=off  T_nominal_value=1  T_nominal_unit=K
  Demux : Demux
  IL : Subsystem
      settings: PortSchema="{\"entries\":[{\"content\":{\"sides\":[{\"content\":{\"connectorIds\":[\"Out1\",\"LConn1\"]},\"type\":\"ConnectorPlacement.EquallySpacedRectSide\",\"uuid\":\"39b7e526-9a68-4c73-9ad6-fd149fea363a\"},{\"content\":{\"connectorIds\":[\"RConn1\"],\"side\":\"RIGHT\"},\"type\":\"ConnectorPlacement.EquallySpacedRectSide\",\"uuid\":\"ee3f62d2-02c4-4290-ad83-c24a9e891d89\"},{\"content\":{\"side\":\"TOP\"},\"type\":\"ConnectorPlacement.EquallySpacedRectSide\",\"uuid\":\"a8618696-d9d3-41f8-b97f-996b903ae337\"}]},\"type\":\"ConnectorPlacement.EquallySpacedConnector\",\"uuid\":\"57ec1f0b-c67f-47bc-9e24-5102208e6cfb\"}],\"packageUris\":[\"http://schema.mathworks.com/mf0/Connector/R2020b\"],\"version\":\"1.0\"}"
      mask Display: disp('I')
  IdealSwitchFastH : ee_lib/Semiconductors & Converters/Ideal Semiconductor Switch  port_option=ee.enum.controlport.ps  Ron=RdsOnFast_SI Ohm  Goff=GdsOffFast_SI 1/Ohm  Vth=VthFast_SI V  diode_param=ee.enum.semiconductors.protectionDiode.nodynamics  diode_Vf=VfFast_SI V  diode_Ron=RdFast_SI Ohm  diode_Goff=GdFast_SI 1/Ohm  diode_C=50e-9 F  diode_iRM=-235 A  diode_iF=300 A  diode_idot=-50 A/us  diode_trr_param=ee.enum.converters.diodetrr.trr_factor  diode_trr_factor=3  diode_trr=15 us  diode_Qrr=1500 s*uA
  IdealSwitchFastL : ee_lib/Semiconductors & Converters/Ideal Semiconductor Switch  port_option=ee.enum.controlport.ps  Ron=RdsOnFast_SI Ohm  Goff=GdsOffFast_SI 1/Ohm  Vth=VthFast_SI V  diode_param=ee.enum.semiconductors.protectionDiode.nodynamics  diode_Vf=VfFast_SI V  diode_Ron=RdFast_SI Ohm  diode_Goff=GdFast_SI 1/Ohm  diode_C=50e-9 F  diode_iRM=-235 A  diode_iF=300 A  diode_idot=-50 A/us  diode_trr_param=ee.enum.converters.diodetrr.trr_factor  diode_trr_factor=3  diode_trr=15 us  diode_Qrr=1500 s*uA
  IdealSwitchSlowtH : ee_lib/Semiconductors & Converters/Ideal Semiconductor Switch  port_option=ee.enum.controlport.ps  Ron=RdsOnSlow_SI Ohm  Goff=GdsOffSlow_SI 1/Ohm  Vth=VthSlow_SI V  diode_param=ee.enum.semiconductors.protectionDiode.nodynamics  diode_Vf=VfSlow_SI V  diode_Ron=RdSlow_SI Ohm  diode_Goff=GdSlow_SI 1/Ohm  diode_C=50e-9 F  diode_iRM=-235 A  diode_iF=300 A  diode_idot=-50 A/us  diode_trr_param=ee.enum.converters.diodetrr.trr_factor  diode_trr_factor=3  diode_trr=15 us  diode_Qrr=1500 s*uA
  IdealSwitchSlowtL : ee_lib/Semiconductors & Converters/Ideal Semiconductor Switch  port_option=ee.enum.controlport.ps  Ron=RdsOnSlow_SI Ohm  Goff=GdsOffSlow_SI 1/Ohm  Vth=VthSlow_SI V  diode_param=ee.enum.semiconductors.protectionDiode.nodynamics  diode_Vf=VfSlow_SI V  diode_Ron=RdSlow_SI Ohm  diode_Goff=GdSlow_SI 1/Ohm  diode_C=50e-9 F  diode_iRM=-235 A  diode_iF=300 A  diode_idot=-50 A/us  diode_trr_param=ee.enum.converters.diodetrr.trr_factor  diode_trr_factor=3  diode_trr=15 us  diode_Qrr=1500 s*uA
  Iout : Subsystem
      mask Display: disp('I')
  Lboost : ee_lib/Passive/Inductor  l=LBoost_SI H  enable_L_tol=ee.enum.toleranceApplication.none  L_tol=20  tol_distribution=ee.enum.toleranceDistribution.uniform  nSigma=4  r=RLboost_SI Ohm  g=1e-9 1/Ohm  enable_operating_limits=ee.enum.enable.no  operating_limit_action=ee.enum.passive.reportOpLim.warn  max_working_current=1 A  power_rating=1 W  i_L_specify=off  i_L_priority=High  i_L=0 A  i_L_nominal_specify=off  i_L_nominal_value=1  i_L_nominal_unit=A
  SL_PS{1..4} (4 alike) : nesl_utility/Simulink-PS Converter  PhysicalDomain=network_engine_domain  SubClassName=ps_input  LeftPortType=input  RightPortType=output  PseudoPeriodic=off  Frequencies=[]  NoiseDistribution=none  NoiseParameters=[]  Unit=1  AffineConversion=off  FilteringAndDerivatives=provide  SimscapeFilterOrder=1  InputFilterTimeConstant=0.001  UdotUserProvided=0
  Vin : Subsystem
      mask Display: disp('V')
  Vout : Subsystem
      settings: PortSchema="{\"entries\":[{\"content\":{\"sides\":[{\"content\":{\"connectorIds\":[\"LConn1\"]},\"type\":\"ConnectorPlacement.EquallySpacedRectSide\",\"uuid\":\"39b7e526-9a68-4c73-9ad6-fd149fea363a\"},{\"content\":{\"connectorIds\":[\"RConn1\",\"Out1\"],\"side\":\"RIGHT\"},\"type\":\"ConnectorPlacement.EquallySpacedRectSide\",\"uuid\":\"ee3f62d2-02c4-4290-ad83-c24a9e891d89\"},{\"content\":{\"side\":\"TOP\"},\"type\":\"ConnectorPlacement.EquallySpacedRectSide\",\"uuid\":\"a8618696-d9d3-41f8-b97f-996b903ae337\"}]},\"type\":\"ConnectorPlacement.EquallySpacedConnector\",\"uuid\":\"57ec1f0b-c67f-47bc-9e24-5102208e6cfb\"}],\"packageUris\":[\"http://schema.mathworks.com/mf0/Connector/R2020b\"],\"version\":\"1.0\"}"
      mask Display: disp('V')
  P : PMIOPort  Side=Left
  N : PMIOPort  Port=2  Side=Left
  + : PMIOPort  Port=3  Side=Right
  - : PMIOPort  Port=4  Side=Right
  Out Bus Element1 : Outport  PortName=meas  Element=IL [A]
  Out Bus Element2 : Outport  PortName=meas  Element=Vout [V]
  Out Bus Element4 : Outport  PortName=meas  Element=Vin [V]
  Out Bus Element5 : Outport  PortName=meas  Element=Iout [A]
  wires:
  Iout/1(I) -> Out Bus Element5/1
  Vin/1(V) -> Out Bus Element4/1
  Vout/1(V) -> Out Bus Element2/1
  IL/1(I) -> Out Bus Element1/1
  [G4] -> SL_PS4/1
  [G3] -> SL_PS3/1
  [G2] -> SL_PS2/1
  [G1] -> SL_PS1/1
  Demux/4 -> [G4]
  Demux/3 -> [G3]
  Demux/2 -> [G2]
  Demux/1 -> [G1]
  G/1 -> Demux/1
  connections:
  Vin/RConn1 -- N/RConn1 -- IdealSwitchSlowtH/RConn2 -- IdealSwitchSlowtL/RConn1
  SL_PS4/RConn1 -- IdealSwitchSlowtL/LConn1
  SL_PS3/RConn1 -- IdealSwitchSlowtH/LConn1
  Co/LConn1 -- Iout/LConn1 -- IdealSwitchSlowtH/RConn1 -- IdealSwitchFastH/RConn1
  IL/RConn1 -- Lboost/LConn1
  +/RConn1 -- Vout/LConn1 -- Iout/RConn1
  -/RConn1 -- Vout/RConn1 -- Co/RConn1 -- IdealSwitchSlowtL/RConn2 -- IdealSwitchFastL/RConn2
  Vin/LConn1 -- P/RConn1 -- IL/LConn1
  SL_PS2/RConn1 -- IdealSwitchFastL/LConn1
  SL_PS1/RConn1 -- IdealSwitchFastH/LConn1
  IdealSwitchFastH/RConn2 -- IdealSwitchFastL/RConn1 -- Lboost/RConn1

== system TotemPoleBoostPFCTestHarnessPlant/PEM Generator/Fast Leg PWM Generator/Ramp Mode/FixedStep ==
  Tsw : Inport
  Initial Ramp Value : InitialCondition  Value=0
  Overshoot Residual : Sum  Inputs=-+
  Period Reached : RelationalOperator  Operator=>  ZeroCross=off
  Time Ramp : DiscreteIntegrator  ExternalReset=rising  InitialConditionSource=external  SampleTime=Ts  ShowStatePort=on  ICPrevOutput=DiscIntNeverNeededParam  ICPrevScaledInput=DiscIntNeverNeededParam
  Unit Rate : Constant
  S : Outport
  wires:
  Initial Ramp Value/1 -> Time Ramp/3
  Overshoot Residual/1 -> Initial Ramp Value/1
  Time Ramp/State -> Overshoot Residual/2, Period Reached/1
  Tsw/1 -> Period Reached/2, Overshoot Residual/1
  Time Ramp/1 -> S/1
  Period Reached/1 -> Time Ramp/2
  Unit Rate/1 -> Time Ramp/1

== system TotemPoleBoostPFCTestHarnessPlant/PEM Generator/Fast Leg PWM Generator/Ramp Mode/VariableStep ==
  Tsw : Inport
  Initial Ramp Value : InitialCondition  Value=0
  Overshoot Residual : Sum  Inputs=-+
  Period Reached : RelationalOperator  Operator=>
  Time Ramp : Integrator  ExternalReset=rising  InitialConditionSource=external  ShowStatePort=on
  Unit Rate : Constant
  S : Outport
  wires:
  Initial Ramp Value/1 -> Time Ramp/3
  Overshoot Residual/1 -> Initial Ramp Value/1
  Time Ramp/State -> Overshoot Residual/2, Period Reached/1
  Tsw/1 -> Period Reached/2, Overshoot Residual/1
  Time Ramp/1 -> S/1
  Period Reached/1 -> Time Ramp/2
  Unit Rate/1 -> Time Ramp/1

== system TotemPoleBoostPFCTestHarnessPlant/PEM Generator/Slow Leg PWM Generator/Ramp Mode/FixedStep ==
  rate : Inport
  Dead Time Timer : DiscreteIntegrator  SampleTime=Ts  LimitOutput=on  UpperSaturationLimit=Tdead  LowerSaturationLimit=0  ICPrevOutput=DiscIntNeverNeededParam  ICPrevScaledInput=DiscIntNeverNeededParam
  S : Outport
  wires:
  Dead Time Timer/1 -> S/1
  rate/1 -> Dead Time Timer/1

== system TotemPoleBoostPFCTestHarnessPlant/PEM Generator/Slow Leg PWM Generator/Ramp Mode/VariableStep ==
  rate : Inport
  Dead Time Timer : Integrator  LimitOutput=on  UpperSaturationLimit=Tdead  LowerSaturationLimit=0
  S : Outport
  wires:
  Dead Time Timer/1 -> S/1
  rate/1 -> Dead Time Timer/1

== system TotemPoleBoostPFCTestHarnessPlant/Totem-Pole Boost PFC/TotemPoleBoostPFCVariant/DetailedModel/FastLeg ==
  G : Inport
  IdealSwitch : Subsystem  VariantControl=IdealSwitch
  SwitchingMOSFETwithThermal : Subsystem  VariantControl=SwitchingMOSFETwithThermal
  Mid : PMIOPort  Side=Left
  DC+ : PMIOPort  Port=2  Side=Right
  DC- : PMIOPort  Port=3  Side=Right

== system TotemPoleBoostPFCTestHarnessPlant/Totem-Pole Boost PFC/TotemPoleBoostPFCVariant/DetailedModel/IL ==
  Current Sensor : fl_lib/Electrical/Electrical Sensors/Current Sensor
  PS-Simulink Converter : nesl_utility/PS-Simulink Converter  PhysicalDomain=network_engine_domain  SubClassName=ps_output  LeftPortType=input  RightPortType=output  PseudoPeriodic=off  Frequencies=[]  VectorFormat=inherit  Unit=inherit  AffineConversion=off
  + : PMIOPort  Side=Left
  - : PMIOPort  Port=2  Side=Right
  I : Outport
  wires:
  PS-Simulink Converter/1 -> I/1
  connections:
  +/RConn1 -- Current Sensor/LConn1
  Current Sensor/RConn2 -- -/RConn1
  Current Sensor/RConn1 -- PS-Simulink Converter/LConn1

== system TotemPoleBoostPFCTestHarnessPlant/Totem-Pole Boost PFC/TotemPoleBoostPFCVariant/DetailedModel/Iout ==
  Current Sensor : fl_lib/Electrical/Electrical Sensors/Current Sensor
  PS-Simulink Converter : nesl_utility/PS-Simulink Converter  PhysicalDomain=network_engine_domain  SubClassName=ps_output  LeftPortType=input  RightPortType=output  PseudoPeriodic=off  Frequencies=[]  VectorFormat=inherit  Unit=inherit  AffineConversion=off
  + : PMIOPort  Side=Left
  - : PMIOPort  Port=2  Side=Right
  I : Outport
  wires:
  PS-Simulink Converter/1 -> I/1
  connections:
  +/RConn1 -- Current Sensor/LConn1
  Current Sensor/RConn2 -- -/RConn1
  Current Sensor/RConn1 -- PS-Simulink Converter/LConn1

== system TotemPoleBoostPFCTestHarnessPlant/Totem-Pole Boost PFC/TotemPoleBoostPFCVariant/DetailedModel/SlowLeg ==
  G : Inport
  Diode : Subsystem  Variant=on  VariantControlMode=label  VariantControl=Diode  LabelModeActiveChoice=IdealDiode
  MOSFET : Subsystem  Variant=on  VariantControlMode=label  VariantControl=MOSFET  LabelModeActiveChoice=SwitchingMOSFETwithThermal
  Thyristor : Subsystem  VariantControl=Thyristor
  DC+ : PMIOPort  Side=Right
  DC- : PMIOPort  Port=2  Side=Right
  Mid : PMIOPort  Port=3  Side=Left

== system TotemPoleBoostPFCTestHarnessPlant/Totem-Pole Boost PFC/TotemPoleBoostPFCVariant/DetailedModel/Vin ==
  PS-Simulink Converter : nesl_utility/PS-Simulink Converter  PhysicalDomain=network_engine_domain  SubClassName=ps_output  LeftPortType=input  RightPortType=output  PseudoPeriodic=off  Frequencies=[]  VectorFormat=inherit  Unit=inherit  AffineConversion=off
  Voltage Sensor : fl_lib/Electrical/Electrical Sensors/Voltage Sensor
  + : PMIOPort  Side=Left
  - : PMIOPort  Port=2  Side=Right
  V : Outport
  wires:
  PS-Simulink Converter/1 -> V/1
  connections:
  +/RConn1 -- Voltage Sensor/LConn1
  Voltage Sensor/RConn2 -- -/RConn1
  Voltage Sensor/RConn1 -- PS-Simulink Converter/LConn1

== system TotemPoleBoostPFCTestHarnessPlant/Totem-Pole Boost PFC/TotemPoleBoostPFCVariant/DetailedModel/Vout ==
  PS-Simulink Converter : nesl_utility/PS-Simulink Converter  PhysicalDomain=network_engine_domain  SubClassName=ps_output  LeftPortType=input  RightPortType=output  PseudoPeriodic=off  Frequencies=[]  VectorFormat=inherit  Unit=inherit  AffineConversion=off
  Voltage Sensor : fl_lib/Electrical/Electrical Sensors/Voltage Sensor
  + : PMIOPort  Side=Left
  - : PMIOPort  Port=2  Side=Right
  V : Outport
  wires:
  PS-Simulink Converter/1 -> V/1
  connections:
  +/RConn1 -- Voltage Sensor/LConn1
  Voltage Sensor/RConn2 -- -/RConn1
  Voltage Sensor/RConn1 -- PS-Simulink Converter/LConn1

== system TotemPoleBoostPFCTestHarnessPlant/Totem-Pole Boost PFC/TotemPoleBoostPFCVariant/SimplifiedModel/IL ==
  Current Sensor : fl_lib/Electrical/Electrical Sensors/Current Sensor
  PS-Simulink Converter : nesl_utility/PS-Simulink Converter  PhysicalDomain=network_engine_domain  SubClassName=ps_output  LeftPortType=input  RightPortType=output  PseudoPeriodic=off  Frequencies=[]  VectorFormat=inherit  Unit=inherit  AffineConversion=off
  + : PMIOPort  Side=Left
  - : PMIOPort  Port=2  Side=Right
  I : Outport
  wires:
  PS-Simulink Converter/1 -> I/1
  connections:
  +/RConn1 -- Current Sensor/LConn1
  Current Sensor/RConn2 -- -/RConn1
  Current Sensor/RConn1 -- PS-Simulink Converter/LConn1

== system TotemPoleBoostPFCTestHarnessPlant/Totem-Pole Boost PFC/TotemPoleBoostPFCVariant/SimplifiedModel/Iout ==
  Current Sensor : fl_lib/Electrical/Electrical Sensors/Current Sensor
  PS-Simulink Converter : nesl_utility/PS-Simulink Converter  PhysicalDomain=network_engine_domain  SubClassName=ps_output  LeftPortType=input  RightPortType=output  PseudoPeriodic=off  Frequencies=[]  VectorFormat=inherit  Unit=inherit  AffineConversion=off
  + : PMIOPort  Side=Left
  - : PMIOPort  Port=2  Side=Right
  I : Outport
  wires:
  PS-Simulink Converter/1 -> I/1
  connections:
  +/RConn1 -- Current Sensor/LConn1
  Current Sensor/RConn2 -- -/RConn1
  Current Sensor/RConn1 -- PS-Simulink Converter/LConn1

== system TotemPoleBoostPFCTestHarnessPlant/Totem-Pole Boost PFC/TotemPoleBoostPFCVariant/SimplifiedModel/Vin ==
  PS-Simulink Converter : nesl_utility/PS-Simulink Converter  PhysicalDomain=network_engine_domain  SubClassName=ps_output  LeftPortType=input  RightPortType=output  PseudoPeriodic=off  Frequencies=[]  VectorFormat=inherit  Unit=inherit  AffineConversion=off
  Voltage Sensor : fl_lib/Electrical/Electrical Sensors/Voltage Sensor
  + : PMIOPort  Side=Left
  - : PMIOPort  Port=2  Side=Right
  V : Outport
  wires:
  PS-Simulink Converter/1 -> V/1
  connections:
  +/RConn1 -- Voltage Sensor/LConn1
  Voltage Sensor/RConn2 -- -/RConn1
  Voltage Sensor/RConn1 -- PS-Simulink Converter/LConn1
